simulink model "NMPC_controller"  (R2023b)
settings: Solver=VariableStepAuto  StartTime=0.0  StopTime=10.0  RelTol=1e-3
libraries: mpclib x1
settings Model: Creator=adwei  LastModifiedBy=adwei

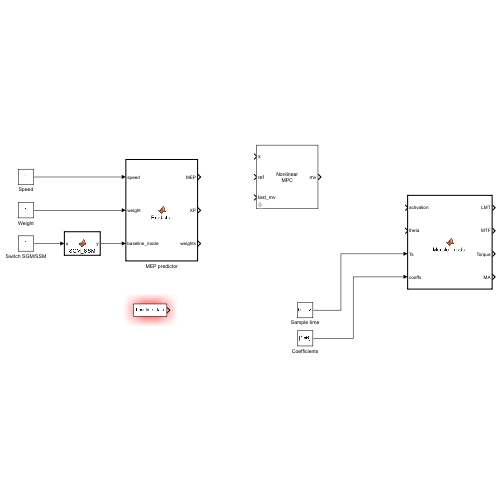
[thumbnail: Simulink's stored preview of the top-level diagram]
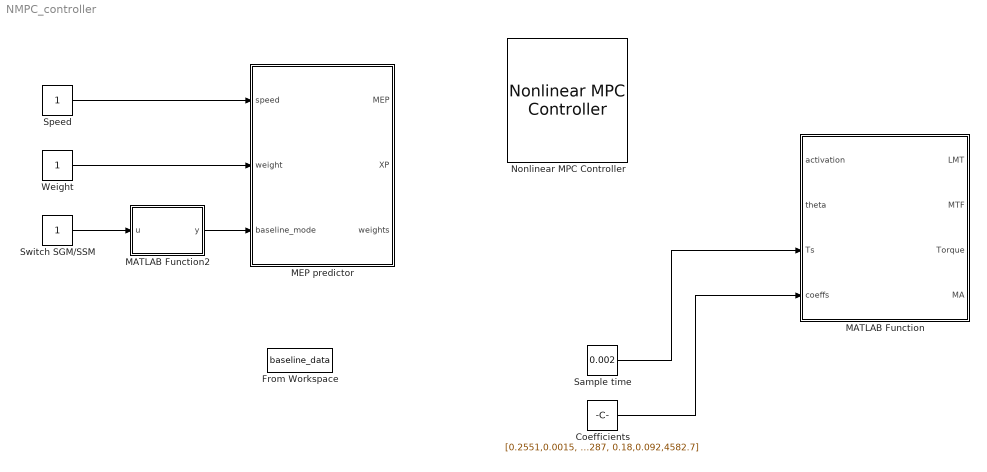
== system NMPC_controller ==
  Coefficients : Constant  Value="[0.2551,0.0015, 0.1287,\t0.18,0.092,4582.7]"  VectorParams1D=off
  From Workspace : FromWorkspace  VariableName=baseline_data
  MATLAB Function : MATLAB Function  TreatAsAtomicUnit=on
  MATLAB Function2 : MATLAB Function  TreatAsAtomicUnit=on
  MEP predictor : MATLAB Function  TreatAsAtomicUnit=on
  Nonlinear MPC Controller : mpclib/Nonlinear MPC Controller  UseObjectTs=on  UseMEX=off  md_enabled=off  mvtarget_enabled=off  param_enabled=off  cost_enabled=off  mvseq_enabled=off  stateseq_enabled=off  ovseq_enabled=off  slack_enabled=off  status_enabled=off  ov_min=off  ov_max=off  mv_min=off  mv_max=off  mvrate_min=off  mvrate_max=off  state_min=off  state_max=off  ov_weight=off  mv_weight=off  mvrate_weight=off  ecr_weight=off  nlp_initialize=off
  Sample time : Constant  Value=0.002
  Speed : Constant
  Switch SGM/SSM : Constant
  Weight : Constant
  wires:
  Coefficients/1 -> MATLAB Function/4(coeffs)
  Sample time/1 -> MATLAB Function/3(Ts)
  MATLAB Function2/1(y) -> MEP predictor/3(baseline_mode)
  Switch SGM/SSM/1 -> MATLAB Function2/1(u)
  Speed/1 -> MEP predictor/1(speed)
  Weight/1 -> MEP predictor/2(weight)

== matlab function NMPC_controller/MEP predictor ==
  data: speed input; MEP output; weight input; XP output; weights output; baseline_mode input
function [MEP, XP, weights] = Predictor(speed, weight, baseline_mode)

[weights, XP, MAP] = MAP_model(speed, weight, baseline_mode, 'baseline_data.mat');
MEP = MAP;

end

== matlab function NMPC_controller/MATLAB Function ==
  data: activation input; LMT output; theta input; Ts input; coeffs input; MTF output; Torque output; MA output
function [LMT, MTF, Torque, MA] = Muscle_model(activation, theta, Ts, coeffs)

  [LMT, MTF, Torque, MA] = Control_model(activation, theta, Ts, coeffs);

end

== matlab function NMPC_controller/MATLAB Function2 ==
  data: u input; y output
function y = SGM_SSM(u)

    % 根据字符变量的值执行不同的操作
    switch mode
        case u
            y = 'SM'; % 模式A对应的输出
        otherwise
            y = 'GM'; % 默认输出
    end
end
